simulink model "slex1"  (R2018b)
settings: Solver=FixedStepAuto  StartTime=0.0  StopTime=10.0  FixedStep=0.01  RelTol=1e-3
settings Model: Creator=19810  LastModifiedBy=19810
settings DataIOCC: InspectSignalLogs=on

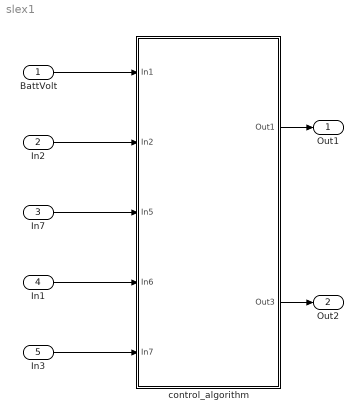
== system slex1 ==
  BattVolt : Inport
  In2 : Inport  Port=2
  In7 : Inport  Port=3
  In1 : Inport  Port=4
  In3 : Inport  Port=5
  control_algorithm : Subsystem
  Out1 : Outport
  Out2 : Outport  Port=2
  wires:
  BattVolt/1 -> control_algorithm/1(In1)
  In2/1 -> control_algorithm/2(In2)
  In7/1 -> control_algorithm/3(In5)
  control_algorithm/1(Out1) -> Out1/1
  In3/1 -> control_algorithm/5(In7)
  In1/1 -> control_algorithm/4(In6)
  control_algorithm/2(Out3) -> Out2/1

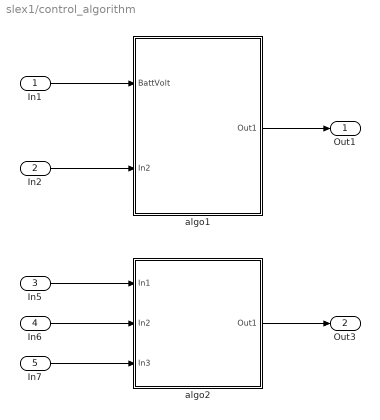
== system slex1/control_algorithm ==
  In1 : Inport
  In2 : Inport  Port=2
  In5 : Inport  Port=3
  In6 : Inport  Port=4
  In7 : Inport  Port=5
  algo1 : Subsystem
  algo2 : Subsystem
  Out1 : Outport
  Out3 : Outport  Port=2
  wires:
  In1/1 -> algo1/1(BattVolt)
  In2/1 -> algo1/2(In2)
  algo1/1(Out1) -> Out1/1
  algo2/1(Out1) -> Out3/1
  In5/1 -> algo2/1(In1)
  In6/1 -> algo2/2(In2)
  In7/1 -> algo2/3(In3)

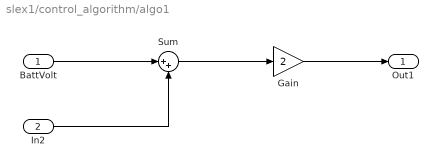
== system slex1/control_algorithm/algo1 ==
  BattVolt : Inport
  In2 : Inport  Port=2
  Gain : Gain  Gain=2
  Sum : Sum  Inputs=|++
  Out1 : Outport
  wires:
  BattVolt/1 -> Sum/1
  In2/1 -> Sum/2
  Sum/1 -> Gain/1
  Gain/1 -> Out1/1

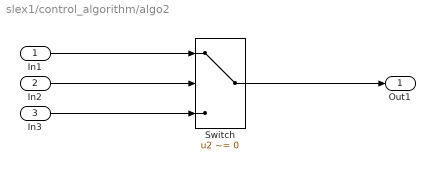
== system slex1/control_algorithm/algo2 ==
  In1 : Inport
  In2 : Inport  Port=2
  In3 : Inport  Port=3
  Switch : Switch  Criteria=u2 ~= 0
  Out1 : Outport
  wires:
  In1/1 -> Switch/1
  In2/1 -> Switch/2
  In3/1 -> Switch/3
  Switch/1 -> Out1/1
